simulink model "EV_HESS_Energy_Management"  (R2025b)
settings: Solver=FixedStepDiscrete  StartTime=0.0  StopTime=400  FixedStep=0.001  RelTol=1e-3
model workspace (MAT data in the model file):
  drive_cycle = [0 1 2 3 4 5 6 7 8 9 10 11 ... (1604 elements, 401x4)]
  hybrid_enabled = 1
  initial_battery_SOC = 0.8
  initial_storage_state = [280.8; 0; 0]
  ml_predictions = [0 1 2 3 4 5 6 7 8 9 10 11 ... (1203 elements, 401x3)]
  plant_parameters_vector = [0.001; 32; 0.001; 0.01; 350; 175.5; 333.45; 100; 0.159375; 0.02; 0.98; 0.000375428571429; 0.0285714285714; 1.2; 0.29; 1.9529; 0.012; 1070; 9.81; 1112.8; 0.85; 0.65; 0; 57.1428571429]
  reference_mode = 1
Description:
  | Electric vehicle hybrid energy storage with analytical, LSTM and GRU current-reference selection. Reduced-order plant with battery-only operation.
settings Model: LastModifiedBy=Dell
settings DataIOCC: SaveOutput=off  SignalLogging=off  SaveTime=off
settings OptimizationCC: BlockReduction=off

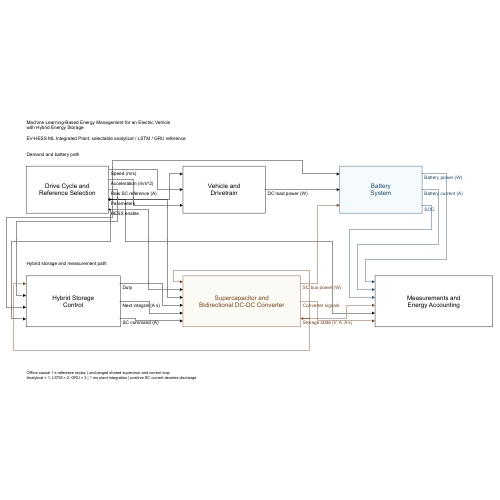
[thumbnail: Simulink's stored preview of the top-level diagram]
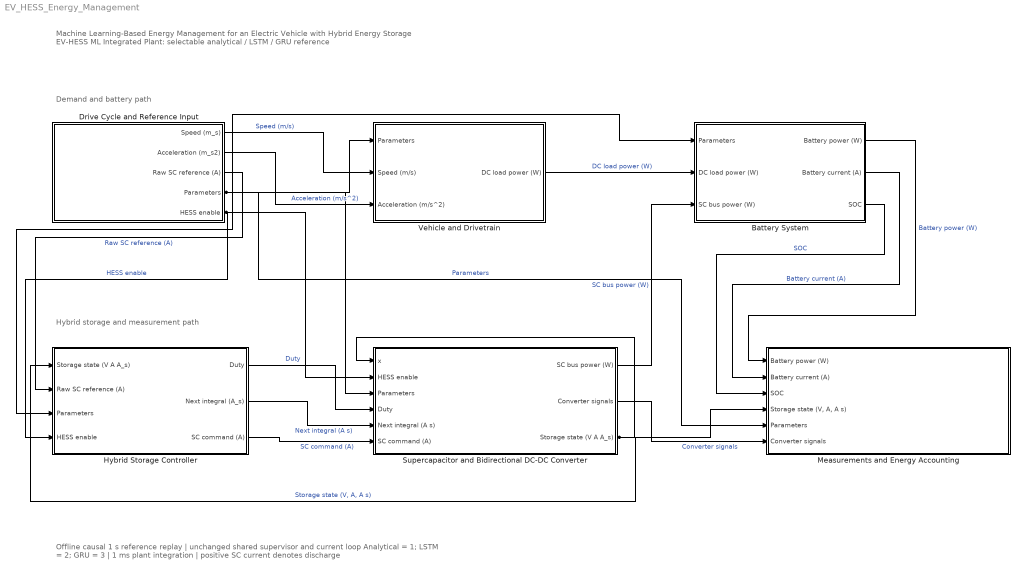
== system EV_HESS_Energy_Management ==
  note: Machine Learning-Based Energy Management for an Electric Vehicle
      | with Hybrid Energy Storage
      |
      | EV-HESS ML Integrated Plant: selectable analytical / LSTM / GRU reference
  note: Offline causal 1 s reference replay | unchanged shared supervisor and current loop
      | Analytical = 1; LSTM = 2; GRU = 3 | 1 ms plant integration | positive SC current denotes discharge
  note: Demand and battery path
  note: Hybrid storage and measurement path
  Battery System : Subsystem
      mask Display: disp(sprintf('Battery\nSystem'))
  Drive Cycle and Reference Input : Subsystem
      mask Display: disp(sprintf('Drive Cycle and\nReference Selection'))
  Hybrid Storage Controller : Subsystem
      mask Display: disp(sprintf('Hybrid Storage\nControl'))
  Measurements and Energy Accounting : Subsystem
      mask Display: disp(sprintf('Measurements and\nEnergy Accounting'))
  Supercapacitor and Bidirectional DC-DC Converter : Subsystem
      mask Display: disp(sprintf('Supercapacitor and\nBidirectional DC-DC Converter'))
  Vehicle and Drivetrain : Subsystem
      mask Display: disp(sprintf('Vehicle and\nDrivetrain'))
  wires:
  Drive Cycle and Reference Input/4(Parameters) -> Measurements and Energy Accounting/5(Parameters), Supercapacitor and Bidirectional DC-DC Converter/3(Parameters), Hybrid Storage Controller/3(Parameters), Battery System/1(Parameters), Vehicle and Drivetrain/1(Parameters)  "Parameters"
  Drive Cycle and Reference Input/5(HESS enable) -> Supercapacitor and Bidirectional DC-DC Converter/2(HESS enable), Hybrid Storage Controller/4(HESS enable)  "HESS enable"
  Drive Cycle and Reference Input/1(Speed (m_s)) -> Vehicle and Drivetrain/2(Speed (m/s))  "Speed (m/s)"
  Drive Cycle and Reference Input/2(Acceleration (m_s2)) -> Vehicle and Drivetrain/3(Acceleration (m/s^2))  "Acceleration (m/s^2)"
  Vehicle and Drivetrain/1(DC load power (W)) -> Battery System/2(DC load power (W))  "DC load power (W)"
  Drive Cycle and Reference Input/3(Raw SC reference (A)) -> Hybrid Storage Controller/2(Raw SC reference (A))  "Raw SC reference (A)"
  Supercapacitor and Bidirectional DC-DC Converter/3(Storage state (V A A_s)) -> Supercapacitor and Bidirectional DC-DC Converter/1(x), Hybrid Storage Controller/1(Storage state (V A A_s)), Measurements and Energy Accounting/4("Storage state (V, A, A s)")  "Storage state (V, A, A s)"
  Hybrid Storage Controller/1(Duty) -> Supercapacitor and Bidirectional DC-DC Converter/4(Duty)  "Duty"
  Hybrid Storage Controller/2(Next integral (A_s)) -> Supercapacitor and Bidirectional DC-DC Converter/5(Next integral (A s))  "Next integral (A s)"
  Hybrid Storage Controller/3(SC command (A)) -> Supercapacitor and Bidirectional DC-DC Converter/6(SC command (A))  "SC command (A)"
  Supercapacitor and Bidirectional DC-DC Converter/1(SC bus power (W)) -> Battery System/3(SC bus power (W))  "SC bus power (W)"
  Battery System/1(Battery power (W)) -> Measurements and Energy Accounting/1(Battery power (W))  "Battery power (W)"
  Battery System/2(Battery current (A)) -> Measurements and Energy Accounting/2(Battery current (A))  "Battery current (A)"
  Battery System/3(SOC) -> Measurements and Energy Accounting/3(SOC)  "SOC"
  Supercapacitor and Bidirectional DC-DC Converter/2(Converter signals) -> Measurements and Energy Accounting/6(Converter signals)  "Converter signals"

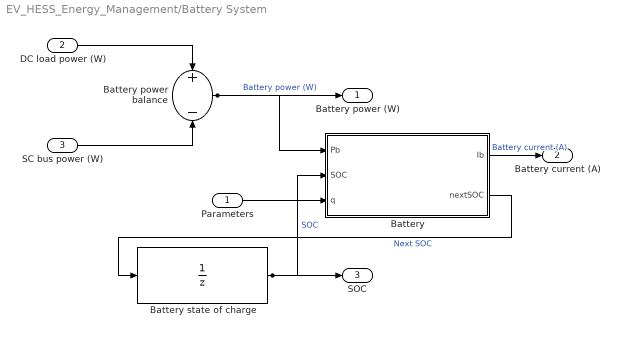
== system EV_HESS_Energy_Management/Battery System ==
  Parameters : Inport
  DC load power (W) : Inport  Port=2
  SC bus power (W) : Inport  Port=3
  Battery : MATLAB Function  TreatAsAtomicUnit=on
  Battery power balance : Sum  Inputs=+-
  Battery state of charge : UnitDelay  InitialCondition=initial_battery_SOC  SampleTime=0.001  HasFrameUpgradeWarning=on
  Battery power (W) : Outport
  Battery current (A) : Outport  Port=2
  SOC : Outport  Port=3
  wires:
  DC load power (W)/1 -> Battery power balance/1
  SC bus power (W)/1 -> Battery power balance/2
  Battery/2(nextSOC) -> Battery state of charge/1  "Next SOC"
  Battery state of charge/1 -> Battery/2(SOC), SOC/1  "SOC"
  Battery power balance/1 -> Battery/1(Pb), Battery power (W)/1  "Battery power (W)"
  Parameters/1 -> Battery/3(q)
  Battery/1(Ib) -> Battery current (A)/1  "Battery current (A)"

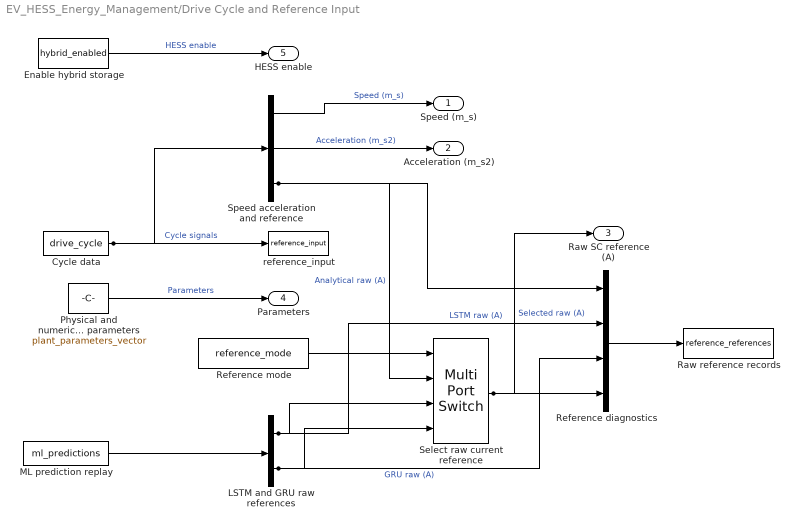
== system EV_HESS_Energy_Management/Drive Cycle and Reference Input ==
  Cycle data : FromWorkspace  VariableName=drive_cycle  SampleTime=0.001  Interpolate=off  OutputAfterFinalValue=Holding final value
  Enable hybrid storage : Constant  Value=hybrid_enabled
  LSTM and GRU raw references : Demux  Outputs=2
  ML prediction replay : FromWorkspace  VariableName=ml_predictions  SampleTime=0.001  Interpolate=off  OutputAfterFinalValue=Holding final value
  Physical and numerical parameters : Constant  Value=plant_parameters_vector
  Raw reference records : ToWorkspace  VariableName=reference_references  SaveFormat=Timeseries  SampleTime=-1
  Reference diagnostics : Mux
  Reference mode : Constant  Value=reference_mode
  Select raw current reference : MultiPortSwitch  SaturateOnIntegerOverflow=off  InputSameDT=off
  Speed acceleration and reference : Demux  Outputs=3
  reference_input : ToWorkspace  VariableName=reference_input  SaveFormat=Timeseries  SampleTime=-1
      mask Display: disp('Input log')
  Speed (m_s) : Outport
  Acceleration (m_s2) : Outport  Port=2
  Raw SC reference (A) : Outport  Port=3
  Parameters : Outport  Port=4
  HESS enable : Outport  Port=5
  wires:
  Cycle data/1 -> Speed acceleration and reference/1, reference_input/1  "Cycle signals"
  Physical and numerical parameters/1 -> Parameters/1  "Parameters"
  Enable hybrid storage/1 -> HESS enable/1  "HESS enable"
  ML prediction replay/1 -> LSTM and GRU raw references/1
  Speed acceleration and reference/1 -> Speed (m_s)/1  "Speed (m_s)"
  Speed acceleration and reference/3 -> Select raw current reference/2, Reference diagnostics/1  "Analytical raw (A)"
  Speed acceleration and reference/2 -> Acceleration (m_s2)/1  "Acceleration (m_s2)"
  Reference mode/1 -> Select raw current reference/1
  LSTM and GRU raw references/1 -> Reference diagnostics/2, Select raw current reference/3  "LSTM raw (A)"
  LSTM and GRU raw references/2 -> Reference diagnostics/3, Select raw current reference/4  "GRU raw (A)"
  Select raw current reference/1 -> Raw SC reference (A)/1, Reference diagnostics/4  "Selected raw (A)"
  Reference diagnostics/1 -> Raw reference records/1

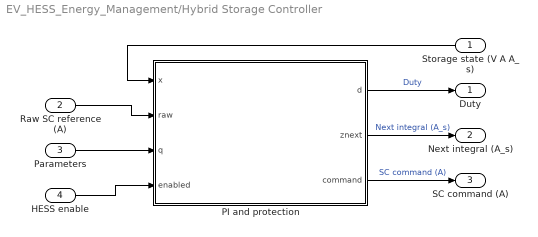
== system EV_HESS_Energy_Management/Hybrid Storage Controller ==
  Storage state (V A A_s) : Inport
  Raw SC reference (A) : Inport  Port=2
  Parameters : Inport  Port=3
  HESS enable : Inport  Port=4
  PI and protection : MATLAB Function  TreatAsAtomicUnit=on
  Duty : Outport
  Next integral (A_s) : Outport  Port=2
  SC command (A) : Outport  Port=3
  wires:
  Storage state (V A A_s)/1 -> PI and protection/1(x)
  Raw SC reference (A)/1 -> PI and protection/2(raw)
  Parameters/1 -> PI and protection/3(q)
  PI and protection/2(znext) -> Next integral (A_s)/1  "Next integral (A_s)"
  HESS enable/1 -> PI and protection/4(enabled)
  PI and protection/1(d) -> Duty/1  "Duty"
  PI and protection/3(command) -> SC command (A)/1  "SC command (A)"

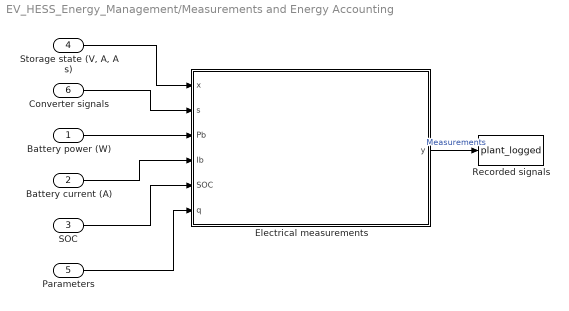
== system EV_HESS_Energy_Management/Measurements and Energy Accounting ==
  Battery power (W) : Inport
  Battery current (A) : Inport  Port=2
  SOC : Inport  Port=3
  "Storage state (V, A, A s)" : Inport  Port=4
  Parameters : Inport  Port=5
  Converter signals : Inport  Port=6
  Electrical measurements : MATLAB Function  TreatAsAtomicUnit=on
  Recorded signals : ToWorkspace  VariableName=plant_logged  SaveFormat=Timeseries  SampleTime=-1
  wires:
  "Storage state (V, A, A s)"/1 -> Electrical measurements/1(x)
  Parameters/1 -> Electrical measurements/6(q)
  SOC/1 -> Electrical measurements/5(SOC)
  Battery current (A)/1 -> Electrical measurements/4(Ib)
  Battery power (W)/1 -> Electrical measurements/3(Pb)
  Converter signals/1 -> Electrical measurements/2(s)
  Electrical measurements/1(y) -> Recorded signals/1  "Measurements"

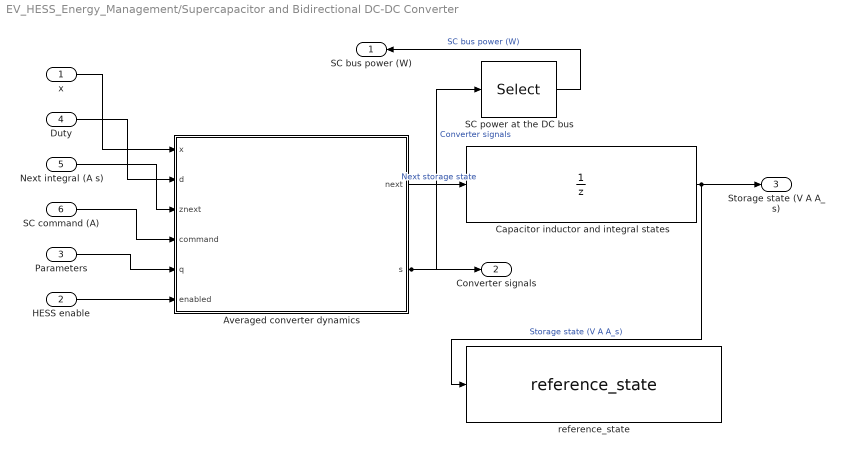
== system EV_HESS_Energy_Management/Supercapacitor and Bidirectional DC-DC Converter ==
  x : Inport
  HESS enable : Inport  Port=2
  Parameters : Inport  Port=3
  Duty : Inport  Port=4
  Next integral (A s) : Inport  Port=5
  SC command (A) : Inport  Port=6
  Averaged converter dynamics : MATLAB Function  TreatAsAtomicUnit=on
  Capacitor inductor and integral states : UnitDelay  InitialCondition=initial_storage_state  SampleTime=0.001  HasFrameUpgradeWarning=on
  SC power at the DC bus : Selector  InputPortWidth=6  IndexOptions=Index vector (dialog)  Indices=3  OutputSizes=1
  reference_state : ToWorkspace  VariableName=reference_state  SaveFormat=Timeseries  SampleTime=-1
  SC bus power (W) : Outport
  Converter signals : Outport  Port=2
  Storage state (V A A_s) : Outport  Port=3
  wires:
  Averaged converter dynamics/2(s) -> SC power at the DC bus/1, Converter signals/1  "Converter signals"
  Capacitor inductor and integral states/1 -> Storage state (V A A_s)/1, reference_state/1  "Storage state (V A A_s)"
  x/1 -> Averaged converter dynamics/1(x)
  Parameters/1 -> Averaged converter dynamics/5(q)
  SC command (A)/1 -> Averaged converter dynamics/4(command)
  Next integral (A s)/1 -> Averaged converter dynamics/3(znext)
  Duty/1 -> Averaged converter dynamics/2(d)
  HESS enable/1 -> Averaged converter dynamics/6(enabled)
  Averaged converter dynamics/1(next) -> Capacitor inductor and integral states/1  "Next storage state"
  SC power at the DC bus/1 -> SC bus power (W)/1  "SC bus power (W)"

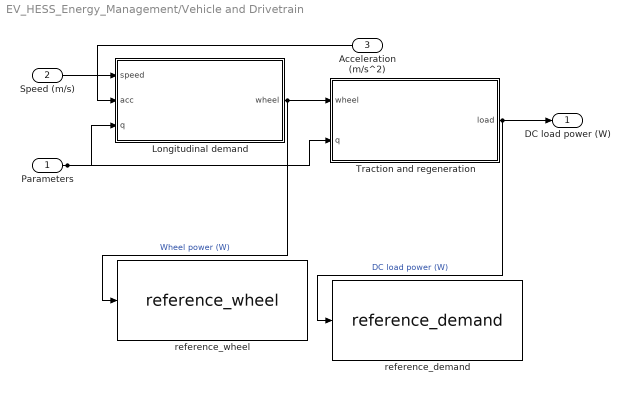
== system EV_HESS_Energy_Management/Vehicle and Drivetrain ==
  Parameters : Inport
  Speed (m/s) : Inport  Port=2
  Acceleration (m/s^2) : Inport  Port=3
  Longitudinal demand : MATLAB Function  TreatAsAtomicUnit=on
  Traction and regeneration : MATLAB Function  TreatAsAtomicUnit=on
  reference_demand : ToWorkspace  VariableName=reference_demand  SaveFormat=Timeseries  SampleTime=-1
  reference_wheel : ToWorkspace  VariableName=reference_wheel  SaveFormat=Timeseries  SampleTime=-1
  DC load power (W) : Outport
  wires:
  Speed (m/s)/1 -> Longitudinal demand/1(speed)
  Acceleration (m/s^2)/1 -> Longitudinal demand/2(acc)
  Parameters/1 -> Traction and regeneration/2(q), Longitudinal demand/3(q)
  Longitudinal demand/1(wheel) -> Traction and regeneration/1(wheel), reference_wheel/1  "Wheel power (W)"
  Traction and regeneration/1(load) -> DC load power (W)/1, reference_demand/1  "DC load power (W)"

== matlab function EV_HESS_Energy_Management/Vehicle and Drivetrain/Traction and regeneration ==
  data: wheel input; load output; q input
function load = plant_sl_drivetrain(wheel,q)
%#codegen
if wheel>=0, load=wheel/q(21); else, load=q(22)*wheel; end
load=load+q(23);
end

== matlab function EV_HESS_Energy_Management/Vehicle and Drivetrain/Longitudinal demand ==
  data: speed input; wheel output; acc input; q input
function wheel = plant_sl_vehicle(speed,acc,q)
%#codegen
Fa=0.5*q(14)*q(15)*q(16)*speed^2;
Fr=q(17)*q(18)*q(19); Fi=q(20)*acc;
wheel=(Fa+Fr+Fi)*speed;
end

== matlab function EV_HESS_Energy_Management/Battery System/Battery ==
  data: Pb input; Ib output; SOC input; q input; nextSOC output
function [Ib,nextSOC] = plant_sl_battery(Pb,SOC,q)
%#codegen
Ib=Pb/q(5); nextSOC=SOC-q(1)*Ib/(3600*q(24));
assert(nextSOC>=0 && nextSOC<=1);
end

== matlab function EV_HESS_Energy_Management/Hybrid Storage Controller/PI and protection ==
  data: x input; d output; raw input; q input; enabled input; znext output; command output
function [d,znext,command] = plant_sl_controller(x,raw,q,enabled)
%#codegen
% Numeric implementation of the documented PI and predictive duty interval.
V=x(1); i=x(2); z=x(3); h=q(1); C=q(2); L=q(3); R=q(4); Vdc=q(5);
if enabled==0
    d=0; znext=0; command=0; return
end
command=min(max(raw,-q(8)),q(8));
if (V<=q(6)+q(9) && command>0) || (V>=q(7)-q(9) && command<0)
    command=0;
end
e=command-i;
rawDuty=V/Vdc-(q(12)*e+q(13)*z);
A=[0,-1/C;1/L,-R/L]; M=eye(2)-h*A/2; N=eye(2)+h*A/2;
alpha=M\(N*[V;i]); beta=M\(h*[0;-Vdc/L]);
vb=[(q(6)-alpha(1))/beta(1),(q(7)-alpha(1))/beta(1)];
ib=[(-q(8)-alpha(2))/beta(2),(q(8)-alpha(2))/beta(2)];
lo=max([q(10),min(vb),min(ib)]); hi=min([q(11),max(vb),max(ib)]);
assert(lo<=hi);
d=min(max(rawDuty,lo),hi);
znext=z;
if abs(d-rawDuty)<=1e-12 || e*(d-rawDuty)<=0
    znext=z+h*e;
end
end

== matlab function EV_HESS_Energy_Management/Supercapacitor and Bidirectional DC-DC Converter/Averaged converter dynamics ==
  data: x input; next output; d input; znext input; command input; q input; enabled input; s output
function [next,s] = plant_sl_converter(x,d,znext,command,q,enabled)
%#codegen
% Implicit midpoint LC transition; s=[i_mid,d,Pbus,loss,command,residual].
if enabled==0
    next=zeros(3,1); s=zeros(6,1); return
end
h=q(1); C=q(2); L=q(3); R=q(4); Vdc=q(5);
A=[0,-1/C;1/L,-R/L]; M=eye(2)-h*A/2; N=eye(2)+h*A/2;
alpha=M\(N*x(1:2)); beta=M\(h*[0;-Vdc/L]);
xn=alpha+beta*d; next=[xn;znext]; mid=(x(1:2)+xn)/2;
Pbus=Vdc*d*mid(2); loss=R*mid(2)^2;
residual=mid(1)*mid(2)-Pbus-L*mid(2)*(xn(2)-x(2))/h-loss;
s=[mid(2);d;Pbus;loss;command;residual];
assert(xn(1)>=q(6)-1e-9 && xn(1)<=q(7)+1e-9);
assert(abs(xn(2))<=q(8)+1e-9);
end

== matlab function EV_HESS_Energy_Management/Measurements and Energy Accounting/Electrical measurements ==
  data: x input; y output; s input; Pb input; Ib input; SOC input; q input
function y = plant_sl_measurements(x,s,Pb,Ib,SOC,q)
%#codegen
% Endpoint states and interval power/current at the current sample.
y=[Pb;Ib;SOC;x(1);x(2);s(1);s(5);s(2);s(3);s(4); ...
    0.5*q(2)*x(1)^2;0.5*q(3)*x(2)^2;s(6)];
end
